simulink library "lib_SecCtrl_MASmsg"  (R2026a)
settings: Solver=VariableStepAuto
undefined symbols (not defined in the file): buses_lf, DiscIntNeverNeededParam, entity, iPs_lf, iQs_lf, last_send, m, Ps_lf, Qs_lf, set_DG_up, set_extra_satur, set_sending_cost, v_buses_mod
libraries: simulink x400, sl_discontinuities x10, eeGeneralControl x5
(part 7 of 12)

== system lib_SecCtrl_MASmsg/MAS messages/ID1/Simulink Function34 ==
  Input1 : Inport
  get_asked : TriggerPort  TriggerType=function-call  IsSimulinkFunction=on  FunctionName=get_asked  FunctionVisibility=scoped  VariantControl=(inherit)
  value : ArgOut  ArgumentName=value
  wires:
  Input1/1 -> value/1

== system lib_SecCtrl_MASmsg/MAS messages/ID1/Simulink Function35 ==
  Input : Inport
  get_extra_satur : TriggerPort  TriggerType=function-call  IsSimulinkFunction=on  FunctionName=get_extra_satur  FunctionVisibility=scoped  VariantControl=(inherit)
  y : ArgOut  ArgumentName=y
  wires:
  Input/1 -> y/1

== system lib_SecCtrl_MASmsg/MAS messages/ID1/Simulink Function36 ==
  Input1 : Inport
  get_Opt : TriggerPort  TriggerType=function-call  IsSimulinkFunction=on  FunctionName=get_Opt  FunctionVisibility=scoped  VariantControl=(inherit)
  value : ArgOut  ArgumentName=value
  wires:
  Input1/1 -> value/1

== system lib_SecCtrl_MASmsg/MAS messages/ID1/Simulink Function37 ==
  set_sending_cost : TriggerPort  TriggerType=function-call  IsSimulinkFunction=on  FunctionName=set_sending_cost  FunctionVisibility=scoped  VariantControl=(inherit)
  u : ArgIn  DisableCoverage=on  ArgumentName=u
  Output : Outport
  wires:
  u/1 -> Output/1

== system lib_SecCtrl_MASmsg/MAS messages/ID1/Simulink Function38 ==
  set_extra_satur : TriggerPort  TriggerType=function-call  IsSimulinkFunction=on  FunctionName=set_extra_satur  FunctionVisibility=scoped  VariantControl=(inherit)
  u : ArgIn  DisableCoverage=on  ArgumentName=u
  Output : Outport
  wires:
  u/1 -> Output/1

== system lib_SecCtrl_MASmsg/MAS messages/ID1/Simulink Function4 ==
  Input2 : Inport
  last_send : TriggerPort  TriggerType=function-call  IsSimulinkFunction=on  FunctionName=last_send  FunctionVisibility=scoped  VariantControl=(inherit)
  u : ArgIn  DisableCoverage=on  ArgumentName=v
  u1 : ArgIn  DisableCoverage=on  Port=2  ArgumentName=omega
  Output : Outport
  Output1 : Outport  Port=2
  time : Outport  Port=3
  wires:
  u/1 -> Output/1  "v"
  u1/1 -> Output1/1  "omega"
  Input2/1 -> time/1  "time"

== system lib_SecCtrl_MASmsg/MAS messages/ID1/Simulink Function5 ==
  send_to : TriggerPort  TriggerType=function-call  IsSimulinkFunction=on  FunctionName=send_to  FunctionVisibility=scoped  VariantControl=(inherit)
  u : ArgIn  DisableCoverage=on  ArgumentName=u
  Output : Outport
  wires:
  u/1 -> Output/1

== system lib_SecCtrl_MASmsg/MAS messages/ID1/Simulink Function6 ==
  Input1 : Inport
  Dest : TriggerPort  TriggerType=function-call  IsSimulinkFunction=on  FunctionName=Dest  FunctionVisibility=scoped  VariantControl=(inherit)
  Dest~ : ArgOut  DisableCoverage=on  ArgumentName=Dest
  wires:
  Input1/1 -> Dest~/1  "Dest"

== system lib_SecCtrl_MASmsg/MAS messages/ID1/Simulink Function7 ==
  set_following : TriggerPort  TriggerType=function-call  IsSimulinkFunction=on  FunctionName=set_following  FunctionVisibility=scoped  VariantControl=(inherit)
  u : ArgIn  DisableCoverage=on  ArgumentName=u
  Output : Outport
  wires:
  u/1 -> Output/1

== system lib_SecCtrl_MASmsg/MAS messages/ID1/Simulink Function8 ==
  type : TriggerPort  TriggerType=function-call  IsSimulinkFunction=on  FunctionName=type  FunctionVisibility=scoped  VariantControl=(inherit)
  Compare To Constant : simulink/Logic and Bit Operations/Compare To Constant  relop=~=  const=0  OutDataTypeStr=boolean  ZeroCross=off
  Send : Send  OutputPortMessageModes=m  ShowEnablePort=on
      settings: InputPortMap=e0,u1
  u : ArgIn  DisableCoverage=on  ArgumentName=u
  type_out : Outport
  trigger : Outport  Port=2
  wires:
  u/1 -> Compare To Constant/1, type_out/1
  Compare To Constant/1 -> Send/1, Send/2
  Send/1 -> trigger/1

== system lib_SecCtrl_MASmsg/MAS messages/ID1/Simulink Function9 ==
  Input1 : Inport
  get_leader : TriggerPort  TriggerType=function-call  IsSimulinkFunction=on  FunctionName=get_leader  FunctionVisibility=scoped  VariantControl=(inherit)
  value : ArgOut  ArgumentName=value
  wires:
  Input1/1 -> value/1

== system lib_SecCtrl_MASmsg/MAS messages/ID1/Subsystem ==
  In1 : Inport
  In3 : Inport  Port=2
  In4 : Inport  Port=3
  AND11 : Logic  IconShape=distinctive  AllPortsSameDT=off  OutDataTypeStr=boolean
  AND9 : Logic  IconShape=distinctive  AllPortsSameDT=off  OutDataTypeStr=boolean
  Compare To Zero : simulink/Logic and Bit Operations/Compare To Zero  relop=>  OutDataTypeStr=boolean
  Compare To Zero1 : simulink/Logic and Bit Operations/Compare To Zero  relop=<  OutDataTypeStr=boolean
  NOT : Logic  Operator=NOT  IconShape=distinctive  AllPortsSameDT=off  OutDataTypeStr=boolean
  OR4 : Logic  Operator=OR  IconShape=distinctive  AllPortsSameDT=off  OutDataTypeStr=boolean
  Relational Operator2 : RelationalOperator  Operator=<  OutDataTypeStr=boolean  RndMeth=Simplest  InputSameDT=off
  Relational Operator3 : RelationalOperator  Operator=>  OutDataTypeStr=boolean  RndMeth=Simplest  InputSameDT=off
  Out1 : Outport
  inf_satur : Outport  Port=2
  wires:
  NOT/1 -> Out1/1
  Compare To Zero/1 -> AND9/2
  Compare To Zero1/1 -> AND11/2
  In3/1 -> Relational Operator3/2, Relational Operator2/2
  Relational Operator3/1 -> AND11/1
  AND11/1 -> OR4/2, inf_satur/1
  In4/1 -> Relational Operator3/1, Relational Operator2/1
  AND9/1 -> OR4/1
  Relational Operator2/1 -> AND9/1
  OR4/1 -> NOT/1
  In1/1 -> Compare To Zero1/1, Compare To Zero/1

== system lib_SecCtrl_MASmsg/MAS messages/ID1/Triggered Subsystem ==
  In1 : Inport
  Trigger : TriggerPort  VariantControl=(inherit)
  Out1 : Outport
  wires:
  In1/1 -> Out1/1

== system lib_SecCtrl_MASmsg/MAS messages/ID1/Triggered Subsystem1 ==
  In1 : Inport
  Trigger : TriggerPort  VariantControl=(inherit)
  Out1 : Outport
  wires:
  In1/1 -> Out1/1

== system lib_SecCtrl_MASmsg/MAS messages/ID1/Triggered Subsystem2 ==
  In1 : Inport
  Trigger : TriggerPort  VariantControl=(inherit)
  Out1 : Outport
  wires:
  In1/1 -> Out1/1

== system lib_SecCtrl_MASmsg/MAS messages/ID1/Triggered Subsystem3 ==
  Trigger : TriggerPort  VariantControl=(inherit)
  One : Constant  OutDataTypeStr=Inherit: Inherit via back propagation
  Send7 : Send  OutputPortMessageModes=m  ShowEnablePort=on
      settings: InputPortMap=e0,u1
  Out1 : Outport
  wires:
  One/1 -> Send7/1, Send7/2
  Send7/1 -> Out1/1

== system lib_SecCtrl_MASmsg/MAS messages/ID1/Triggered Subsystem4 ==
  In1 : Inport
  Trigger : TriggerPort  VariantControl=(inherit)
  Out1 : Outport
  wires:
  In1/1 -> Out1/1

== system lib_SecCtrl_MASmsg/MAS messages/ID1/Triggered Subsystem5 ==
  In1 : Inport
  Trigger : TriggerPort  TriggerType=falling  VariantControl=(inherit)
  Constant : Constant
  IC : InitialCondition  Value=0
  Out1 : Outport
  Output : Outport  Port=2
  wires:
  IC/1 -> Output/1
  Constant/1 -> IC/1
  In1/1 -> Out1/1

== system lib_SecCtrl_MASmsg/MAS messages/ID1/ramp ==
  connected : Inport
  time : Inport  Port=2
  Clock5 : Clock
      settings: DisableCoverage=on
  Gain : Gain  Gain=0.05
  Product : Product
  Sum6 : Sum  DisableCoverage=on  Inputs=|+-  InputSameDT=on  SaturateOnIntegerOverflow=on  OutDataTypeStr=Inherit: Same as first input
  Out1 : Outport
  wires:
  Clock5/1 -> Sum6/1
  time/1 -> Sum6/2
  Sum6/1 -> Product/2
  Gain/1 -> Out1/1
  Product/1 -> Gain/1
  connected/1 -> Product/1

== system lib_SecCtrl_MASmsg/MAS messages/ID1/time ==
  time : Inport
  Trigger : TriggerPort  VariantControl=(inherit)
  Out1 : Outport
  wires:
  time/1 -> Out1/1

== system lib_SecCtrl_MASmsg/MAS messages/ID2/Compare to last ==
  Output : Inport
  In4 : Inport  Port=2
  In1 : Inport  Port=3
  Output1 : Inport  Port=4
  time_last : Inport  Port=5
  com : Inport  Port=6
  AND : Logic  Inputs=3  IconShape=distinctive  AllPortsSameDT=off  OutDataTypeStr=boolean
  Abs : Abs  ZeroCross=off  SaturateOnIntegerOverflow=off
  Abs1 : Abs  ZeroCross=off  SaturateOnIntegerOverflow=off
  Clock1 : Clock
  Compare To Constant1 : simulink/Logic and Bit Operations/Compare To Constant  relop=>  const=1  OutDataTypeStr=boolean  ZeroCross=off
  Compare To Constant2 : simulink/Logic and Bit Operations/Compare To Constant  relop=>  const=1e-2  OutDataTypeStr=boolean  ZeroCross=off
  Gain : Gain  Gain=1e2
  Gain1 : Gain  Gain=1e2
  Send1 : Send  OutputPortMessageModes=m  ShowEnablePort=on
      settings: InputPortMap=e0,u1
  Sum : Sum  Inputs=|+-
  Sum1 : Sum  Inputs=|+-
  Sum2 : Sum  Inputs=|++
  Sum5 : Sum  Inputs=|+-
  Trigger : Outport
  wires:
  com/1 -> AND/3
  Gain1/1 -> Sum2/2
  Gain/1 -> Sum2/1
  Compare To Constant1/1 -> AND/1
  Sum2/1 -> Compare To Constant1/1
  Abs1/1 -> Gain1/1
  Compare To Constant2/1 -> AND/2
  Clock1/1 -> Sum1/1  "time"
  time_last/1 -> Sum1/2  "time_last"
  Sum1/1 -> Compare To Constant2/1
  AND/1 -> Send1/2, Send1/1
  In4/1 -> Sum5/2  "last_omega"
  Sum5/1 -> Abs1/1
  Abs/1 -> Gain/1
  Sum/1 -> Abs/1
  Send1/1 -> Trigger/1
  Output1/1 -> Sum5/1  "omega"
  In1/1 -> Sum/1  "v"
  Output/1 -> Sum/2  "last_v"

== system lib_SecCtrl_MASmsg/MAS messages/ID2/Send to neighbor ==
  note: 1) Add Subsystem or Model blocks as valid variant choices.
      | 2) You cannot connect blocks at this level. At simulation, connectivity is automatically
      | determined, based on the active variant and port name matching.
  Message : Inport
  five : Subsystem  VariantControl=five
  four : Subsystem  VariantControl=four
  one : Subsystem  VariantControl=one
  three : Subsystem  VariantControl=three
  two : Subsystem  VariantControl=two

== system lib_SecCtrl_MASmsg/MAS messages/ID2/Send to neighbor1 ==
  note: 1) Add Subsystem or Model blocks as valid variant choices.
      | 2) You cannot connect blocks at this level. At simulation, connectivity is automatically
      | determined, based on the active variant and port name matching.
  Message : Inport
  five : Subsystem  VariantControl=five
  four : Subsystem  VariantControl=four
  one : Subsystem  VariantControl=one
  three : Subsystem  VariantControl=three
  two : Subsystem  VariantControl=two

== system lib_SecCtrl_MASmsg/MAS messages/ID2/Send to neighbor2 ==
  note: 1) Add Subsystem or Model blocks as valid variant choices.
      | 2) You cannot connect blocks at this level. At simulation, connectivity is automatically
      | determined, based on the active variant and port name matching.
  Message : Inport
  five : Subsystem  VariantControl=five
  four : Subsystem  VariantControl=four
  one : Subsystem  VariantControl=one
  three : Subsystem  VariantControl=three
  two : Subsystem  VariantControl=two

== system lib_SecCtrl_MASmsg/MAS messages/ID2/Simulink Function ==
  Input : Inport
  get_cost : TriggerPort  TriggerType=function-call  IsSimulinkFunction=on  FunctionName=get_cost  FunctionVisibility=scoped  VariantControl=(inherit)
  y : ArgOut  DisableCoverage=on  ArgumentName=y
  wires:
  Input/1 -> y/1

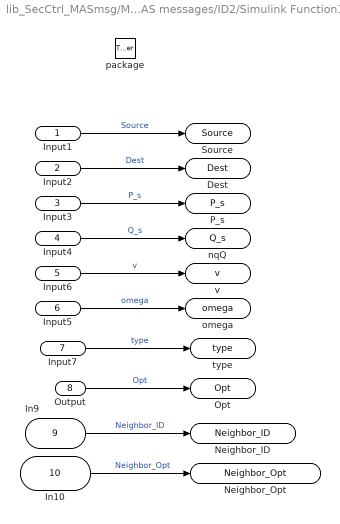
== system lib_SecCtrl_MASmsg/MAS messages/ID2/Simulink Function1 ==
  Input1 : Inport
  Input2 : Inport  Port=2
  Input3 : Inport  Port=3
  Input4 : Inport  Port=4
  Input6 : Inport  Port=5
  Input5 : Inport  Port=6
  Input7 : Inport  Port=7
  Output : Inport  Port=8
  In9 : Inport  Port=9
  In10 : Inport  Port=10
  package : TriggerPort  TriggerType=function-call  IsSimulinkFunction=on  FunctionName=package  FunctionVisibility=scoped  VariantControl=(inherit)
  Source : ArgOut  DisableCoverage=on  ArgumentName=Source
  Dest : ArgOut  DisableCoverage=on  Port=2  ArgumentName=Dest
  P_s : ArgOut  DisableCoverage=on  Port=3  ArgumentName=P_s
  nqQ : ArgOut  DisableCoverage=on  Port=4  ArgumentName=Q_s
  v : ArgOut  DisableCoverage=on  Port=5  ArgumentName=v
  omega : ArgOut  DisableCoverage=on  Port=6  ArgumentName=omega
  type : ArgOut  DisableCoverage=on  Port=7  ArgumentName=type
  Opt : ArgOut  Port=8  ArgumentName=Opt
  Neighbor_ID : ArgOut  Port=9  ArgumentName=Neighbor_ID
  Neighbor_Opt : ArgOut  Port=10  ArgumentName=Neighbor_Opt
  wires:
  In9/1 -> Neighbor_ID/1  "Neighbor_ID"
  In10/1 -> Neighbor_Opt/1  "Neighbor_Opt"
  Output/1 -> Opt/1  "Opt"
  Input7/1 -> type/1  "type"
  Input5/1 -> omega/1  "omega"
  Input6/1 -> v/1  "v"
  Input4/1 -> nqQ/1  "Q_s"
  Input3/1 -> P_s/1  "P_s"
  Input2/1 -> Dest/1  "Dest"
  Input1/1 -> Source/1  "Source"

== system lib_SecCtrl_MASmsg/MAS messages/ID2/Simulink Function10 ==
  set_leader : TriggerPort  TriggerType=function-call  IsSimulinkFunction=on  FunctionName=set_leader  FunctionVisibility=scoped  VariantControl=(inherit)
  u : ArgIn  DisableCoverage=on  ArgumentName=u
  Output : Outport
  wires:
  u/1 -> Output/1

== system lib_SecCtrl_MASmsg/MAS messages/ID2/Simulink Function11 ==
  Input1 : Inport
  get_sending : TriggerPort  TriggerType=function-call  IsSimulinkFunction=on  FunctionName=get_sending  FunctionVisibility=scoped  VariantControl=(inherit)
  value : ArgOut  ArgumentName=value
  wires:
  Input1/1 -> value/1

== system lib_SecCtrl_MASmsg/MAS messages/ID2/Simulink Function12 ==
  set_sending : TriggerPort  TriggerType=function-call  IsSimulinkFunction=on  FunctionName=set_sending  FunctionVisibility=scoped  VariantControl=(inherit)
  u : ArgIn  DisableCoverage=on  ArgumentName=u
  Output : Outport
  wires:
  u/1 -> Output/1

== system lib_SecCtrl_MASmsg/MAS messages/ID2/Simulink Function13 ==
  Input1 : Inport
  get_type : TriggerPort  TriggerType=function-call  IsSimulinkFunction=on  FunctionName=get_type  FunctionVisibility=scoped  VariantControl=(inherit)
  value : ArgOut  ArgumentName=type
  wires:
  Input1/1 -> value/1  "type"

== system lib_SecCtrl_MASmsg/MAS messages/ID2/Simulink Function14 ==
  set_cost_info : TriggerPort  TriggerType=function-call  IsSimulinkFunction=on  FunctionName=set_cost_info  FunctionVisibility=scoped  VariantControl=(inherit)
  cost : ArgIn  ArgumentName=cost
  Output : Outport
  wires:
  cost/1 -> Output/1

== system lib_SecCtrl_MASmsg/MAS messages/ID2/Simulink Function15 ==
  set_DG_up : TriggerPort  TriggerType=function-call  IsSimulinkFunction=on  FunctionName=set_DG_up  FunctionVisibility=scoped  VariantControl=(inherit)
  u : ArgIn  DisableCoverage=on  ArgumentName=u
  Output : Outport
  wires:
  u/1 -> Output/1

== system lib_SecCtrl_MASmsg/MAS messages/ID2/Simulink Function16 ==
  Input1 : Inport
  get_DG_up : TriggerPort  TriggerType=function-call  IsSimulinkFunction=on  FunctionName=get_DG_up  FunctionVisibility=scoped  VariantControl=(inherit)
  value : ArgOut  OutDataTypeStr=boolean  ArgumentName=value
  wires:
  Input1/1 -> value/1

== system lib_SecCtrl_MASmsg/MAS messages/ID2/Simulink Function17 ==
  set_neigh_ID : TriggerPort  TriggerType=function-call  IsSimulinkFunction=on  FunctionName=set_neigh_ID  FunctionVisibility=scoped  VariantControl=(inherit)
  u : ArgIn  DisableCoverage=on  ArgumentName=u
  Output : Outport
  wires:
  u/1 -> Output/1

== system lib_SecCtrl_MASmsg/MAS messages/ID2/Simulink Function18 ==
  Input1 : Inport
  get_neigh_ID : TriggerPort  TriggerType=function-call  IsSimulinkFunction=on  FunctionName=get_neigh_ID  FunctionVisibility=scoped  VariantControl=(inherit)
  value : ArgOut  ArgumentName=value
  wires:
  Input1/1 -> value/1

== system lib_SecCtrl_MASmsg/MAS messages/ID2/Simulink Function19 ==
  set_neigh_Opt : TriggerPort  TriggerType=function-call  IsSimulinkFunction=on  FunctionName=set_neigh_Opt  FunctionVisibility=scoped  VariantControl=(inherit)
  u : ArgIn  DisableCoverage=on  ArgumentName=u
  Output : Outport
  wires:
  u/1 -> Output/1

== system lib_SecCtrl_MASmsg/MAS messages/ID2/Simulink Function2 ==
  unpackage : TriggerPort  TriggerType=function-call  IsSimulinkFunction=on  FunctionName=unpackage  FunctionVisibility=scoped  VariantControl=(inherit)
  IC1 : InitialCondition
  IC2 : InitialCondition
  IC3 : InitialCondition  Value=v_buses_mod(buses_lf(IDnumber))
  IC4 : InitialCondition
  mpP~ : ArgIn  ArgumentName=P_s
  nqQ~ : ArgIn  Port=2  ArgumentName=Q_s
  v : ArgIn  Port=3  ArgumentName=v
  omega : ArgIn  Port=4  ArgumentName=omega
  Output2 : Outport
  Output3 : Outport  Port=2
  Output4 : Outport  Port=3
  Output5 : Outport  Port=4
  wires:
  omega/1 -> IC4/1  "omega"
  v/1 -> IC3/1  "v"
  nqQ~/1 -> IC2/1  "Q_s"
  mpP~/1 -> IC1/1  "P_s"
  IC1/1 -> Output2/1
  IC2/1 -> Output3/1
  IC4/1 -> Output5/1
  IC3/1 -> Output4/1

== system lib_SecCtrl_MASmsg/MAS messages/ID2/Simulink Function20 ==
  Input1 : Inport
  get_neigh_Opt : TriggerPort  TriggerType=function-call  IsSimulinkFunction=on  FunctionName=get_neigh_Opt  FunctionVisibility=scoped  VariantControl=(inherit)
  value : ArgOut  ArgumentName=value
  wires:
  Input1/1 -> value/1

== system lib_SecCtrl_MASmsg/MAS messages/ID2/Simulink Function21 ==
  set_sum_neigh_left : TriggerPort  TriggerType=function-call  IsSimulinkFunction=on  FunctionName=set_sum_neigh_left  FunctionVisibility=scoped  VariantControl=(inherit)
  u : ArgIn  DisableCoverage=on  ArgumentName=u
  Output : Outport
  wires:
  u/1 -> Output/1

== system lib_SecCtrl_MASmsg/MAS messages/ID2/Simulink Function22 ==
  set_Opt : TriggerPort  TriggerType=function-call  IsSimulinkFunction=on  FunctionName=set_Opt  FunctionVisibility=scoped  VariantControl=(inherit)
  u : ArgIn  DisableCoverage=on  ArgumentName=u
  Output : Outport
  wires:
  u/1 -> Output/1

== system lib_SecCtrl_MASmsg/MAS messages/ID2/Simulink Function23 ==
  Input1 : Inport
  get_sum_neigh_left : TriggerPort  TriggerType=function-call  IsSimulinkFunction=on  FunctionName=get_sum_neigh_left  FunctionVisibility=scoped  VariantControl=(inherit)
  value : ArgOut  ArgumentName=value
  wires:
  Input1/1 -> value/1  "sum_neigh_left"

== system lib_SecCtrl_MASmsg/MAS messages/ID2/Simulink Function24 ==
  set_decision_turn : TriggerPort  TriggerType=function-call  IsSimulinkFunction=on  FunctionName=set_decision_turn  FunctionVisibility=scoped  VariantControl=(inherit)
  u : ArgIn  DisableCoverage=on  ArgumentName=u
  Output : Outport
  wires:
  u/1 -> Output/1

== system lib_SecCtrl_MASmsg/MAS messages/ID2/Simulink Function25 ==
  Input1 : Inport
  get_ID : TriggerPort  TriggerType=function-call  IsSimulinkFunction=on  FunctionName=get_ID  FunctionVisibility=scoped  VariantControl=(inherit)
  value : ArgOut  ArgumentName=value
  wires:
  Input1/1 -> value/1

== system lib_SecCtrl_MASmsg/MAS messages/ID2/Simulink Function26 ==
  set_Neighbor_ID : TriggerPort  TriggerType=function-call  IsSimulinkFunction=on  FunctionName=set_Neighbor_ID  FunctionVisibility=scoped  VariantControl=(inherit)
  u : ArgIn  DisableCoverage=on  ArgumentName=u
  Output : Outport
  wires:
  u/1 -> Output/1

== system lib_SecCtrl_MASmsg/MAS messages/ID2/Simulink Function27 ==
  set_original_Opt : TriggerPort  TriggerType=function-call  IsSimulinkFunction=on  FunctionName=set_original_Opt  FunctionVisibility=scoped  VariantControl=(inherit)
  u : ArgIn  DisableCoverage=on  ArgumentName=u
  Output : Outport
  wires:
  u/1 -> Output/1

== system lib_SecCtrl_MASmsg/MAS messages/ID2/Simulink Function28 ==
  set_Neighbor_Opt : TriggerPort  TriggerType=function-call  IsSimulinkFunction=on  FunctionName=set_Neighbor_Opt  FunctionVisibility=scoped  VariantControl=(inherit)
  u : ArgIn  DisableCoverage=on  ArgumentName=u
  Output : Outport
  wires:
  u/1 -> Output/1

== system lib_SecCtrl_MASmsg/MAS messages/ID2/Simulink Function29 ==
  Input1 : Inport
  get_original_Opt : TriggerPort  TriggerType=function-call  IsSimulinkFunction=on  FunctionName=get_original_Opt  FunctionVisibility=scoped  VariantControl=(inherit)
  value : ArgOut  ArgumentName=value
  wires:
  Input1/1 -> value/1

== system lib_SecCtrl_MASmsg/MAS messages/ID2/Simulink Function3 ==
  Input1 : Inport
  get_following : TriggerPort  TriggerType=function-call  IsSimulinkFunction=on  FunctionName=get_following  FunctionVisibility=scoped  VariantControl=(inherit)
  value : ArgOut  ArgumentName=value
  wires:
  Input1/1 -> value/1

== system lib_SecCtrl_MASmsg/MAS messages/ID2/Simulink Function30 ==
  set_original_ID : TriggerPort  TriggerType=function-call  IsSimulinkFunction=on  FunctionName=set_original_ID  FunctionVisibility=scoped  VariantControl=(inherit)
  u : ArgIn  DisableCoverage=on  ArgumentName=u
  Output : Outport
  wires:
  u/1 -> Output/1

== system lib_SecCtrl_MASmsg/MAS messages/ID2/Simulink Function31 ==
  Input1 : Inport
  get_original_ID : TriggerPort  TriggerType=function-call  IsSimulinkFunction=on  FunctionName=get_original_ID  FunctionVisibility=scoped  VariantControl=(inherit)
  value : ArgOut  ArgumentName=value
  wires:
  Input1/1 -> value/1

== system lib_SecCtrl_MASmsg/MAS messages/ID2/Simulink Function32 ==
  set_asked : TriggerPort  TriggerType=function-call  IsSimulinkFunction=on  FunctionName=set_asked  FunctionVisibility=scoped  VariantControl=(inherit)
  u : ArgIn  DisableCoverage=on  ArgumentName=u
  Output : Outport
  wires:
  u/1 -> Output/1

== system lib_SecCtrl_MASmsg/MAS messages/ID2/Simulink Function33 ==
  Input : Inport
  get_cost_P : TriggerPort  TriggerType=function-call  IsSimulinkFunction=on  FunctionName=get_cost_P  FunctionVisibility=scoped  VariantControl=(inherit)
  y : ArgOut  DisableCoverage=on  ArgumentName=y
  wires:
  Input/1 -> y/1

== system lib_SecCtrl_MASmsg/MAS messages/ID2/Simulink Function34 ==
  Input1 : Inport
  get_asked : TriggerPort  TriggerType=function-call  IsSimulinkFunction=on  FunctionName=get_asked  FunctionVisibility=scoped  VariantControl=(inherit)
  value : ArgOut  ArgumentName=value
  wires:
  Input1/1 -> value/1

== system lib_SecCtrl_MASmsg/MAS messages/ID2/Simulink Function35 ==
  Input : Inport
  get_extra_satur : TriggerPort  TriggerType=function-call  IsSimulinkFunction=on  FunctionName=get_extra_satur  FunctionVisibility=scoped  VariantControl=(inherit)
  y : ArgOut  ArgumentName=y
  wires:
  Input/1 -> y/1

== system lib_SecCtrl_MASmsg/MAS messages/ID2/Simulink Function36 ==
  Input1 : Inport
  get_Opt : TriggerPort  TriggerType=function-call  IsSimulinkFunction=on  FunctionName=get_Opt  FunctionVisibility=scoped  VariantControl=(inherit)
  value : ArgOut  ArgumentName=value
  wires:
  Input1/1 -> value/1

== system lib_SecCtrl_MASmsg/MAS messages/ID2/Simulink Function37 ==
  set_sending_cost : TriggerPort  TriggerType=function-call  IsSimulinkFunction=on  FunctionName=set_sending_cost  FunctionVisibility=scoped  VariantControl=(inherit)
  u : ArgIn  DisableCoverage=on  ArgumentName=u
  Output : Outport
  wires:
  u/1 -> Output/1

== system lib_SecCtrl_MASmsg/MAS messages/ID2/Simulink Function38 ==
  set_extra_satur : TriggerPort  TriggerType=function-call  IsSimulinkFunction=on  FunctionName=set_extra_satur  FunctionVisibility=scoped  VariantControl=(inherit)
  u : ArgIn  DisableCoverage=on  ArgumentName=u
  Output : Outport
  wires:
  u/1 -> Output/1

== system lib_SecCtrl_MASmsg/MAS messages/ID2/Simulink Function4 ==
  Input2 : Inport
  last_send : TriggerPort  TriggerType=function-call  IsSimulinkFunction=on  FunctionName=last_send  FunctionVisibility=scoped  VariantControl=(inherit)
  u : ArgIn  DisableCoverage=on  ArgumentName=v
  u1 : ArgIn  DisableCoverage=on  Port=2  ArgumentName=omega
  Output : Outport
  Output1 : Outport  Port=2
  time : Outport  Port=3
  wires:
  Input2/1 -> time/1  "time"
  u1/1 -> Output1/1  "omega"
  u/1 -> Output/1  "v"

== system lib_SecCtrl_MASmsg/MAS messages/ID2/Simulink Function5 ==
  send_to : TriggerPort  TriggerType=function-call  IsSimulinkFunction=on  FunctionName=send_to  FunctionVisibility=scoped  VariantControl=(inherit)
  u : ArgIn  DisableCoverage=on  ArgumentName=u
  Output : Outport
  wires:
  u/1 -> Output/1

== system lib_SecCtrl_MASmsg/MAS messages/ID2/Simulink Function6 ==
  Input1 : Inport
  Dest : TriggerPort  TriggerType=function-call  IsSimulinkFunction=on  FunctionName=Dest  FunctionVisibility=scoped  VariantControl=(inherit)
  Dest~ : ArgOut  DisableCoverage=on  ArgumentName=Dest
  wires:
  Input1/1 -> Dest~/1  "Dest"

== system lib_SecCtrl_MASmsg/MAS messages/ID2/Simulink Function7 ==
  set_following : TriggerPort  TriggerType=function-call  IsSimulinkFunction=on  FunctionName=set_following  FunctionVisibility=scoped  VariantControl=(inherit)
  u : ArgIn  DisableCoverage=on  ArgumentName=u
  Output : Outport
  wires:
  u/1 -> Output/1

== system lib_SecCtrl_MASmsg/MAS messages/ID2/Simulink Function8 ==
  type : TriggerPort  TriggerType=function-call  IsSimulinkFunction=on  FunctionName=type  FunctionVisibility=scoped  VariantControl=(inherit)
  Compare To Constant : simulink/Logic and Bit Operations/Compare To Constant  relop=~=  const=0  OutDataTypeStr=boolean  ZeroCross=off
  Send : Send  OutputPortMessageModes=m  ShowEnablePort=on
      settings: InputPortMap=e0,u1
  u : ArgIn  DisableCoverage=on  ArgumentName=u
  type_out : Outport
  trigger : Outport  Port=2
  wires:
  Send/1 -> trigger/1
  Compare To Constant/1 -> Send/2, Send/1
  u/1 -> type_out/1, Compare To Constant/1

== system lib_SecCtrl_MASmsg/MAS messages/ID2/Simulink Function9 ==
  Input1 : Inport
  get_leader : TriggerPort  TriggerType=function-call  IsSimulinkFunction=on  FunctionName=get_leader  FunctionVisibility=scoped  VariantControl=(inherit)
  value : ArgOut  ArgumentName=value
  wires:
  Input1/1 -> value/1

== system lib_SecCtrl_MASmsg/MAS messages/ID2/Subsystem ==
  In1 : Inport
  In3 : Inport  Port=2
  In4 : Inport  Port=3
  AND11 : Logic  IconShape=distinctive  AllPortsSameDT=off  OutDataTypeStr=boolean
  AND9 : Logic  IconShape=distinctive  AllPortsSameDT=off  OutDataTypeStr=boolean
  Compare To Zero : simulink/Logic and Bit Operations/Compare To Zero  relop=>  OutDataTypeStr=boolean
  Compare To Zero1 : simulink/Logic and Bit Operations/Compare To Zero  relop=<  OutDataTypeStr=boolean
  NOT : Logic  Operator=NOT  IconShape=distinctive  AllPortsSameDT=off  OutDataTypeStr=boolean
  OR4 : Logic  Operator=OR  IconShape=distinctive  AllPortsSameDT=off  OutDataTypeStr=boolean
  Relational Operator2 : RelationalOperator  Operator=<  OutDataTypeStr=boolean  RndMeth=Simplest  InputSameDT=off
  Relational Operator3 : RelationalOperator  Operator=>  OutDataTypeStr=boolean  RndMeth=Simplest  InputSameDT=off
  Out1 : Outport
  inf_satur : Outport  Port=2
  wires:
  In1/1 -> Compare To Zero/1, Compare To Zero1/1
  OR4/1 -> NOT/1
  Relational Operator2/1 -> AND9/1
  AND9/1 -> OR4/1
  In4/1 -> Relational Operator2/1, Relational Operator3/1
  AND11/1 -> inf_satur/1, OR4/2
  Relational Operator3/1 -> AND11/1
  In3/1 -> Relational Operator2/2, Relational Operator3/2
  Compare To Zero1/1 -> AND11/2
  Compare To Zero/1 -> AND9/2
  NOT/1 -> Out1/1

== system lib_SecCtrl_MASmsg/MAS messages/ID2/Triggered Subsystem ==
  In1 : Inport
  Trigger : TriggerPort  VariantControl=(inherit)
  Out1 : Outport
  wires:
  In1/1 -> Out1/1

== system lib_SecCtrl_MASmsg/MAS messages/ID2/Triggered Subsystem1 ==
  In1 : Inport
  Trigger : TriggerPort  VariantControl=(inherit)
  Out1 : Outport
  wires:
  In1/1 -> Out1/1

== system lib_SecCtrl_MASmsg/MAS messages/ID2/Triggered Subsystem2 ==
  In1 : Inport
  Trigger : TriggerPort  VariantControl=(inherit)
  Out1 : Outport
  wires:
  In1/1 -> Out1/1

== system lib_SecCtrl_MASmsg/MAS messages/ID2/Triggered Subsystem3 ==
  Trigger : TriggerPort  VariantControl=(inherit)
  One : Constant  OutDataTypeStr=Inherit: Inherit via back propagation
  Send7 : Send  OutputPortMessageModes=m  ShowEnablePort=on
      settings: InputPortMap=e0,u1
  Out1 : Outport
  wires:
  Send7/1 -> Out1/1
  One/1 -> Send7/2, Send7/1

== system lib_SecCtrl_MASmsg/MAS messages/ID2/Triggered Subsystem4 ==
  In1 : Inport
  Trigger : TriggerPort  VariantControl=(inherit)
  Out1 : Outport
  wires:
  In1/1 -> Out1/1

== system lib_SecCtrl_MASmsg/MAS messages/ID2/Triggered Subsystem5 ==
  In1 : Inport
  Trigger : TriggerPort  TriggerType=falling  VariantControl=(inherit)
  Constant : Constant
  IC : InitialCondition  Value=0
  Out1 : Outport
  Output : Outport  Port=2
  wires:
  In1/1 -> Out1/1
  Constant/1 -> IC/1
  IC/1 -> Output/1

== system lib_SecCtrl_MASmsg/MAS messages/ID2/ramp ==
  connected : Inport
  time : Inport  Port=2
  Clock5 : Clock
      settings: DisableCoverage=on
  Gain : Gain  Gain=0.05
  Product : Product
  Sum6 : Sum  DisableCoverage=on  Inputs=|+-  InputSameDT=on  SaturateOnIntegerOverflow=on  OutDataTypeStr=Inherit: Same as first input
  Out1 : Outport
  wires:
  connected/1 -> Product/1
  Product/1 -> Gain/1
  Gain/1 -> Out1/1
  Sum6/1 -> Product/2
  time/1 -> Sum6/2
  Clock5/1 -> Sum6/1

== system lib_SecCtrl_MASmsg/MAS messages/ID2/time ==
  time : Inport
  Trigger : TriggerPort  VariantControl=(inherit)
  Out1 : Outport
  wires:
  time/1 -> Out1/1

== system lib_SecCtrl_MASmsg/MAS messages/ID3/Compare to last ==
  Output : Inport
  In4 : Inport  Port=2
  In1 : Inport  Port=3
  Output1 : Inport  Port=4
  time_last : Inport  Port=5
  com : Inport  Port=6
  AND : Logic  Inputs=3  IconShape=distinctive  AllPortsSameDT=off  OutDataTypeStr=boolean
  Abs : Abs  ZeroCross=off  SaturateOnIntegerOverflow=off
  Abs1 : Abs  ZeroCross=off  SaturateOnIntegerOverflow=off
  Clock1 : Clock
  Compare To Constant1 : simulink/Logic and Bit Operations/Compare To Constant  relop=>  const=1  OutDataTypeStr=boolean  ZeroCross=off
  Compare To Constant2 : simulink/Logic and Bit Operations/Compare To Constant  relop=>  const=1e-2  OutDataTypeStr=boolean  ZeroCross=off
  Gain : Gain  Gain=1e2
  Gain1 : Gain  Gain=1e2
  Send1 : Send  OutputPortMessageModes=m  ShowEnablePort=on
      settings: InputPortMap=e0,u1
  Sum : Sum  Inputs=|+-
  Sum1 : Sum  Inputs=|+-
  Sum2 : Sum  Inputs=|++
  Sum5 : Sum  Inputs=|+-
  Trigger : Outport
  wires:
  com/1 -> AND/3
  Gain1/1 -> Sum2/2
  Gain/1 -> Sum2/1
  Compare To Constant1/1 -> AND/1
  Sum2/1 -> Compare To Constant1/1
  Abs1/1 -> Gain1/1
  Compare To Constant2/1 -> AND/2
  Clock1/1 -> Sum1/1  "time"
  time_last/1 -> Sum1/2  "time_last"
  Sum1/1 -> Compare To Constant2/1
  AND/1 -> Send1/2, Send1/1
  In4/1 -> Sum5/2  "last_omega"
  Sum5/1 -> Abs1/1
  Abs/1 -> Gain/1
  Sum/1 -> Abs/1
  Send1/1 -> Trigger/1
  Output1/1 -> Sum5/1  "omega"
  In1/1 -> Sum/1  "v"
  Output/1 -> Sum/2  "last_v"

== system lib_SecCtrl_MASmsg/MAS messages/ID3/Send to neighbor ==
  note: 1) Add Subsystem or Model blocks as valid variant choices.
      | 2) You cannot connect blocks at this level. At simulation, connectivity is automatically
      | determined, based on the active variant and port name matching.
  Message : Inport
  five : Subsystem  VariantControl=five
  four : Subsystem  VariantControl=four
  one : Subsystem  VariantControl=one
  three : Subsystem  VariantControl=three
  two : Subsystem  VariantControl=two

== system lib_SecCtrl_MASmsg/MAS messages/ID3/Send to neighbor1 ==
  note: 1) Add Subsystem or Model blocks as valid variant choices.
      | 2) You cannot connect blocks at this level. At simulation, connectivity is automatically
      | determined, based on the active variant and port name matching.
  Message : Inport
  five : Subsystem  VariantControl=five
  four : Subsystem  VariantControl=four
  one : Subsystem  VariantControl=one
  three : Subsystem  VariantControl=three
  two : Subsystem  VariantControl=two

== system lib_SecCtrl_MASmsg/MAS messages/ID3/Send to neighbor2 ==
  note: 1) Add Subsystem or Model blocks as valid variant choices.
      | 2) You cannot connect blocks at this level. At simulation, connectivity is automatically
      | determined, based on the active variant and port name matching.
  Message : Inport
  five : Subsystem  VariantControl=five
  four : Subsystem  VariantControl=four
  one : Subsystem  VariantControl=one
  three : Subsystem  VariantControl=three
  two : Subsystem  VariantControl=two

== system lib_SecCtrl_MASmsg/MAS messages/ID3/Simulink Function ==
  Input : Inport
  get_cost : TriggerPort  TriggerType=function-call  IsSimulinkFunction=on  FunctionName=get_cost  FunctionVisibility=scoped  VariantControl=(inherit)
  y : ArgOut  DisableCoverage=on  ArgumentName=y
  wires:
  Input/1 -> y/1

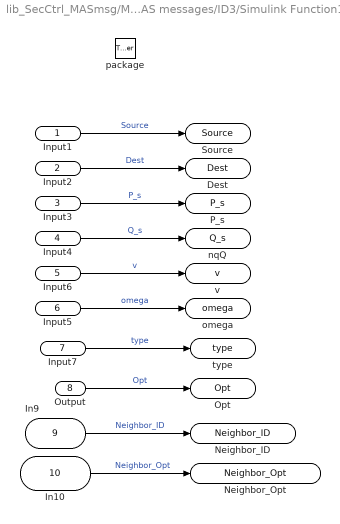
== system lib_SecCtrl_MASmsg/MAS messages/ID3/Simulink Function1 ==
  Input1 : Inport
  Input2 : Inport  Port=2
  Input3 : Inport  Port=3
  Input4 : Inport  Port=4
  Input6 : Inport  Port=5
  Input5 : Inport  Port=6
  Input7 : Inport  Port=7
  Output : Inport  Port=8
  In9 : Inport  Port=9
  In10 : Inport  Port=10
  package : TriggerPort  TriggerType=function-call  IsSimulinkFunction=on  FunctionName=package  FunctionVisibility=scoped  VariantControl=(inherit)
  Source : ArgOut  DisableCoverage=on  ArgumentName=Source
  Dest : ArgOut  DisableCoverage=on  Port=2  ArgumentName=Dest
  P_s : ArgOut  DisableCoverage=on  Port=3  ArgumentName=P_s
  nqQ : ArgOut  DisableCoverage=on  Port=4  ArgumentName=Q_s
  v : ArgOut  DisableCoverage=on  Port=5  ArgumentName=v
  omega : ArgOut  DisableCoverage=on  Port=6  ArgumentName=omega
  type : ArgOut  DisableCoverage=on  Port=7  ArgumentName=type
  Opt : ArgOut  Port=8  ArgumentName=Opt
  Neighbor_ID : ArgOut  Port=9  ArgumentName=Neighbor_ID
  Neighbor_Opt : ArgOut  Port=10  ArgumentName=Neighbor_Opt
  wires:
  In9/1 -> Neighbor_ID/1  "Neighbor_ID"
  In10/1 -> Neighbor_Opt/1  "Neighbor_Opt"
  Output/1 -> Opt/1  "Opt"
  Input7/1 -> type/1  "type"
  Input5/1 -> omega/1  "omega"
  Input6/1 -> v/1  "v"
  Input4/1 -> nqQ/1  "Q_s"
  Input3/1 -> P_s/1  "P_s"
  Input2/1 -> Dest/1  "Dest"
  Input1/1 -> Source/1  "Source"

== system lib_SecCtrl_MASmsg/MAS messages/ID3/Simulink Function10 ==
  set_leader : TriggerPort  TriggerType=function-call  IsSimulinkFunction=on  FunctionName=set_leader  FunctionVisibility=scoped  VariantControl=(inherit)
  u : ArgIn  DisableCoverage=on  ArgumentName=u
  Output : Outport
  wires:
  u/1 -> Output/1

== system lib_SecCtrl_MASmsg/MAS messages/ID3/Simulink Function11 ==
  Input1 : Inport
  get_sending : TriggerPort  TriggerType=function-call  IsSimulinkFunction=on  FunctionName=get_sending  FunctionVisibility=scoped  VariantControl=(inherit)
  value : ArgOut  ArgumentName=value
  wires:
  Input1/1 -> value/1

== system lib_SecCtrl_MASmsg/MAS messages/ID3/Simulink Function12 ==
  set_sending : TriggerPort  TriggerType=function-call  IsSimulinkFunction=on  FunctionName=set_sending  FunctionVisibility=scoped  VariantControl=(inherit)
  u : ArgIn  DisableCoverage=on  ArgumentName=u
  Output : Outport
  wires:
  u/1 -> Output/1

== system lib_SecCtrl_MASmsg/MAS messages/ID3/Simulink Function13 ==
  Input1 : Inport
  get_type : TriggerPort  TriggerType=function-call  IsSimulinkFunction=on  FunctionName=get_type  FunctionVisibility=scoped  VariantControl=(inherit)
  value : ArgOut  ArgumentName=type
  wires:
  Input1/1 -> value/1  "type"

== system lib_SecCtrl_MASmsg/MAS messages/ID3/Simulink Function14 ==
  set_cost_info : TriggerPort  TriggerType=function-call  IsSimulinkFunction=on  FunctionName=set_cost_info  FunctionVisibility=scoped  VariantControl=(inherit)
  cost : ArgIn  ArgumentName=cost
  Output : Outport
  wires:
  cost/1 -> Output/1

== system lib_SecCtrl_MASmsg/MAS messages/ID3/Simulink Function15 ==
  set_DG_up : TriggerPort  TriggerType=function-call  IsSimulinkFunction=on  FunctionName=set_DG_up  FunctionVisibility=scoped  VariantControl=(inherit)
  u : ArgIn  DisableCoverage=on  ArgumentName=u
  Output : Outport
  wires:
  u/1 -> Output/1

== system lib_SecCtrl_MASmsg/MAS messages/ID3/Simulink Function16 ==
  Input1 : Inport
  get_DG_up : TriggerPort  TriggerType=function-call  IsSimulinkFunction=on  FunctionName=get_DG_up  FunctionVisibility=scoped  VariantControl=(inherit)
  value : ArgOut  OutDataTypeStr=boolean  ArgumentName=value
  wires:
  Input1/1 -> value/1

== system lib_SecCtrl_MASmsg/MAS messages/ID3/Simulink Function17 ==
  set_neigh_ID : TriggerPort  TriggerType=function-call  IsSimulinkFunction=on  FunctionName=set_neigh_ID  FunctionVisibility=scoped  VariantControl=(inherit)
  u : ArgIn  DisableCoverage=on  ArgumentName=u
  Output : Outport
  wires:
  u/1 -> Output/1

== system lib_SecCtrl_MASmsg/MAS messages/ID3/Simulink Function18 ==
  Input1 : Inport
  get_neigh_ID : TriggerPort  TriggerType=function-call  IsSimulinkFunction=on  FunctionName=get_neigh_ID  FunctionVisibility=scoped  VariantControl=(inherit)
  value : ArgOut  ArgumentName=value
  wires:
  Input1/1 -> value/1

== system lib_SecCtrl_MASmsg/MAS messages/ID3/Simulink Function19 ==
  set_neigh_Opt : TriggerPort  TriggerType=function-call  IsSimulinkFunction=on  FunctionName=set_neigh_Opt  FunctionVisibility=scoped  VariantControl=(inherit)
  u : ArgIn  DisableCoverage=on  ArgumentName=u
  Output : Outport
  wires:
  u/1 -> Output/1

== system lib_SecCtrl_MASmsg/MAS messages/ID3/Simulink Function2 ==
  unpackage : TriggerPort  TriggerType=function-call  IsSimulinkFunction=on  FunctionName=unpackage  FunctionVisibility=scoped  VariantControl=(inherit)
  IC1 : InitialCondition
  IC2 : InitialCondition
  IC3 : InitialCondition  Value=v_buses_mod(buses_lf(IDnumber))
  IC4 : InitialCondition
  mpP~ : ArgIn  ArgumentName=P_s
  nqQ~ : ArgIn  Port=2  ArgumentName=Q_s
  v : ArgIn  Port=3  ArgumentName=v
  omega : ArgIn  Port=4  ArgumentName=omega
  Output2 : Outport
  Output3 : Outport  Port=2
  Output4 : Outport  Port=3
  Output5 : Outport  Port=4
  wires:
  omega/1 -> IC4/1  "omega"
  v/1 -> IC3/1  "v"
  nqQ~/1 -> IC2/1  "Q_s"
  mpP~/1 -> IC1/1  "P_s"
  IC1/1 -> Output2/1
  IC2/1 -> Output3/1
  IC4/1 -> Output5/1
  IC3/1 -> Output4/1

== system lib_SecCtrl_MASmsg/MAS messages/ID3/Simulink Function20 ==
  Input1 : Inport
  get_neigh_Opt : TriggerPort  TriggerType=function-call  IsSimulinkFunction=on  FunctionName=get_neigh_Opt  FunctionVisibility=scoped  VariantControl=(inherit)
  value : ArgOut  ArgumentName=value
  wires:
  Input1/1 -> value/1

== system lib_SecCtrl_MASmsg/MAS messages/ID3/Simulink Function21 ==
  set_sum_neigh_left : TriggerPort  TriggerType=function-call  IsSimulinkFunction=on  FunctionName=set_sum_neigh_left  FunctionVisibility=scoped  VariantControl=(inherit)
  u : ArgIn  DisableCoverage=on  ArgumentName=u
  Output : Outport
  wires:
  u/1 -> Output/1

== system lib_SecCtrl_MASmsg/MAS messages/ID3/Simulink Function22 ==
  set_Opt : TriggerPort  TriggerType=function-call  IsSimulinkFunction=on  FunctionName=set_Opt  FunctionVisibility=scoped  VariantControl=(inherit)
  u : ArgIn  DisableCoverage=on  ArgumentName=u
  Output : Outport
  wires:
  u/1 -> Output/1

== system lib_SecCtrl_MASmsg/MAS messages/ID3/Simulink Function23 ==
  Input1 : Inport
  get_sum_neigh_left : TriggerPort  TriggerType=function-call  IsSimulinkFunction=on  FunctionName=get_sum_neigh_left  FunctionVisibility=scoped  VariantControl=(inherit)
  value : ArgOut  ArgumentName=value
  wires:
  Input1/1 -> value/1  "sum_neigh_left"

== system lib_SecCtrl_MASmsg/MAS messages/ID3/Simulink Function24 ==
  set_decision_turn : TriggerPort  TriggerType=function-call  IsSimulinkFunction=on  FunctionName=set_decision_turn  FunctionVisibility=scoped  VariantControl=(inherit)
  u : ArgIn  DisableCoverage=on  ArgumentName=u
  Output : Outport
  wires:
  u/1 -> Output/1

== system lib_SecCtrl_MASmsg/MAS messages/ID3/Simulink Function25 ==
  Input1 : Inport
  get_ID : TriggerPort  TriggerType=function-call  IsSimulinkFunction=on  FunctionName=get_ID  FunctionVisibility=scoped  VariantControl=(inherit)
  value : ArgOut  ArgumentName=value
  wires:
  Input1/1 -> value/1

== system lib_SecCtrl_MASmsg/MAS messages/ID3/Simulink Function26 ==
  set_Neighbor_ID : TriggerPort  TriggerType=function-call  IsSimulinkFunction=on  FunctionName=set_Neighbor_ID  FunctionVisibility=scoped  VariantControl=(inherit)
  u : ArgIn  DisableCoverage=on  ArgumentName=u
  Output : Outport
  wires:
  u/1 -> Output/1

== system lib_SecCtrl_MASmsg/MAS messages/ID3/Simulink Function27 ==
  set_original_Opt : TriggerPort  TriggerType=function-call  IsSimulinkFunction=on  FunctionName=set_original_Opt  FunctionVisibility=scoped  VariantControl=(inherit)
  u : ArgIn  DisableCoverage=on  ArgumentName=u
  Output : Outport
  wires:
  u/1 -> Output/1

== system lib_SecCtrl_MASmsg/MAS messages/ID3/Simulink Function28 ==
  set_Neighbor_Opt : TriggerPort  TriggerType=function-call  IsSimulinkFunction=on  FunctionName=set_Neighbor_Opt  FunctionVisibility=scoped  VariantControl=(inherit)
  u : ArgIn  DisableCoverage=on  ArgumentName=u
  Output : Outport
  wires:
  u/1 -> Output/1

== system lib_SecCtrl_MASmsg/MAS messages/ID3/Simulink Function29 ==
  Input1 : Inport
  get_original_Opt : TriggerPort  TriggerType=function-call  IsSimulinkFunction=on  FunctionName=get_original_Opt  FunctionVisibility=scoped  VariantControl=(inherit)
  value : ArgOut  ArgumentName=value
  wires:
  Input1/1 -> value/1

== system lib_SecCtrl_MASmsg/MAS messages/ID3/Simulink Function3 ==
  Input1 : Inport
  get_following : TriggerPort  TriggerType=function-call  IsSimulinkFunction=on  FunctionName=get_following  FunctionVisibility=scoped  VariantControl=(inherit)
  value : ArgOut  ArgumentName=value
  wires:
  Input1/1 -> value/1

== system lib_SecCtrl_MASmsg/MAS messages/ID3/Simulink Function30 ==
  set_original_ID : TriggerPort  TriggerType=function-call  IsSimulinkFunction=on  FunctionName=set_original_ID  FunctionVisibility=scoped  VariantControl=(inherit)
  u : ArgIn  DisableCoverage=on  ArgumentName=u
  Output : Outport
  wires:
  u/1 -> Output/1

== system lib_SecCtrl_MASmsg/MAS messages/ID3/Simulink Function31 ==
  Input1 : Inport
  get_original_ID : TriggerPort  TriggerType=function-call  IsSimulinkFunction=on  FunctionName=get_original_ID  FunctionVisibility=scoped  VariantControl=(inherit)
  value : ArgOut  ArgumentName=value
  wires:
  Input1/1 -> value/1

== system lib_SecCtrl_MASmsg/MAS messages/ID3/Simulink Function32 ==
  set_asked : TriggerPort  TriggerType=function-call  IsSimulinkFunction=on  FunctionName=set_asked  FunctionVisibility=scoped  VariantControl=(inherit)
  u : ArgIn  DisableCoverage=on  ArgumentName=u
  Output : Outport
  wires:
  u/1 -> Output/1

== system lib_SecCtrl_MASmsg/MAS messages/ID3/Simulink Function33 ==
  Input : Inport
  get_cost_P : TriggerPort  TriggerType=function-call  IsSimulinkFunction=on  FunctionName=get_cost_P  FunctionVisibility=scoped  VariantControl=(inherit)
  y : ArgOut  DisableCoverage=on  ArgumentName=y
  wires:
  Input/1 -> y/1

== system lib_SecCtrl_MASmsg/MAS messages/ID3/Simulink Function34 ==
  Input1 : Inport
  get_asked : TriggerPort  TriggerType=function-call  IsSimulinkFunction=on  FunctionName=get_asked  FunctionVisibility=scoped  VariantControl=(inherit)
  value : ArgOut  ArgumentName=value
  wires:
  Input1/1 -> value/1

== system lib_SecCtrl_MASmsg/MAS messages/ID3/Simulink Function35 ==
  Input : Inport
  get_extra_satur : TriggerPort  TriggerType=function-call  IsSimulinkFunction=on  FunctionName=get_extra_satur  FunctionVisibility=scoped  VariantControl=(inherit)
  y : ArgOut  ArgumentName=y
  wires:
  Input/1 -> y/1

== system lib_SecCtrl_MASmsg/MAS messages/ID3/Simulink Function36 ==
  Input1 : Inport
  get_Opt : TriggerPort  TriggerType=function-call  IsSimulinkFunction=on  FunctionName=get_Opt  FunctionVisibility=scoped  VariantControl=(inherit)
  value : ArgOut  ArgumentName=value
  wires:
  Input1/1 -> value/1

== system lib_SecCtrl_MASmsg/MAS messages/ID3/Simulink Function37 ==
  set_sending_cost : TriggerPort  TriggerType=function-call  IsSimulinkFunction=on  FunctionName=set_sending_cost  FunctionVisibility=scoped  VariantControl=(inherit)
  u : ArgIn  DisableCoverage=on  ArgumentName=u
  Output : Outport
  wires:
  u/1 -> Output/1

== system lib_SecCtrl_MASmsg/MAS messages/ID3/Simulink Function38 ==
  set_extra_satur : TriggerPort  TriggerType=function-call  IsSimulinkFunction=on  FunctionName=set_extra_satur  FunctionVisibility=scoped  VariantControl=(inherit)
  u : ArgIn  DisableCoverage=on  ArgumentName=u
  Output : Outport
  wires:
  u/1 -> Output/1

== system lib_SecCtrl_MASmsg/MAS messages/ID3/Simulink Function4 ==
  Input2 : Inport
  last_send : TriggerPort  TriggerType=function-call  IsSimulinkFunction=on  FunctionName=last_send  FunctionVisibility=scoped  VariantControl=(inherit)
  u : ArgIn  DisableCoverage=on  ArgumentName=v
  u1 : ArgIn  DisableCoverage=on  Port=2  ArgumentName=omega
  Output : Outport
  Output1 : Outport  Port=2
  time : Outport  Port=3
  wires:
  Input2/1 -> time/1  "time"
  u1/1 -> Output1/1  "omega"
  u/1 -> Output/1  "v"

== system lib_SecCtrl_MASmsg/MAS messages/ID3/Simulink Function5 ==
  send_to : TriggerPort  TriggerType=function-call  IsSimulinkFunction=on  FunctionName=send_to  FunctionVisibility=scoped  VariantControl=(inherit)
  u : ArgIn  DisableCoverage=on  ArgumentName=u
  Output : Outport
  wires:
  u/1 -> Output/1

== system lib_SecCtrl_MASmsg/MAS messages/ID3/Simulink Function6 ==
  Input1 : Inport
  Dest : TriggerPort  TriggerType=function-call  IsSimulinkFunction=on  FunctionName=Dest  FunctionVisibility=scoped  VariantControl=(inherit)
  Dest~ : ArgOut  DisableCoverage=on  ArgumentName=Dest
  wires:
  Input1/1 -> Dest~/1  "Dest"

== system lib_SecCtrl_MASmsg/MAS messages/ID3/Simulink Function7 ==
  set_following : TriggerPort  TriggerType=function-call  IsSimulinkFunction=on  FunctionName=set_following  FunctionVisibility=scoped  VariantControl=(inherit)
  u : ArgIn  DisableCoverage=on  ArgumentName=u
  Output : Outport
  wires:
  u/1 -> Output/1

== system lib_SecCtrl_MASmsg/MAS messages/ID3/Simulink Function8 ==
  type : TriggerPort  TriggerType=function-call  IsSimulinkFunction=on  FunctionName=type  FunctionVisibility=scoped  VariantControl=(inherit)
  Compare To Constant : simulink/Logic and Bit Operations/Compare To Constant  relop=~=  const=0  OutDataTypeStr=boolean  ZeroCross=off
  Send : Send  OutputPortMessageModes=m  ShowEnablePort=on
      settings: InputPortMap=e0,u1
  u : ArgIn  DisableCoverage=on  ArgumentName=u
  type_out : Outport
  trigger : Outport  Port=2
  wires:
  Send/1 -> trigger/1
  Compare To Constant/1 -> Send/2, Send/1
  u/1 -> type_out/1, Compare To Constant/1

== system lib_SecCtrl_MASmsg/MAS messages/ID3/Simulink Function9 ==
  Input1 : Inport
  get_leader : TriggerPort  TriggerType=function-call  IsSimulinkFunction=on  FunctionName=get_leader  FunctionVisibility=scoped  VariantControl=(inherit)
  value : ArgOut  ArgumentName=value
  wires:
  Input1/1 -> value/1

== system lib_SecCtrl_MASmsg/MAS messages/ID3/Subsystem ==
  In1 : Inport
  In3 : Inport  Port=2
  In4 : Inport  Port=3
  AND11 : Logic  IconShape=distinctive  AllPortsSameDT=off  OutDataTypeStr=boolean
  AND9 : Logic  IconShape=distinctive  AllPortsSameDT=off  OutDataTypeStr=boolean
  Compare To Zero : simulink/Logic and Bit Operations/Compare To Zero  relop=>  OutDataTypeStr=boolean
  Compare To Zero1 : simulink/Logic and Bit Operations/Compare To Zero  relop=<  OutDataTypeStr=boolean
  NOT : Logic  Operator=NOT  IconShape=distinctive  AllPortsSameDT=off  OutDataTypeStr=boolean
  OR4 : Logic  Operator=OR  IconShape=distinctive  AllPortsSameDT=off  OutDataTypeStr=boolean
  Relational Operator2 : RelationalOperator  Operator=<  OutDataTypeStr=boolean  RndMeth=Simplest  InputSameDT=off
  Relational Operator3 : RelationalOperator  Operator=>  OutDataTypeStr=boolean  RndMeth=Simplest  InputSameDT=off
  Out1 : Outport
  inf_satur : Outport  Port=2
  wires:
  In1/1 -> Compare To Zero/1, Compare To Zero1/1
  OR4/1 -> NOT/1
  Relational Operator2/1 -> AND9/1
  AND9/1 -> OR4/1
  In4/1 -> Relational Operator2/1, Relational Operator3/1
  AND11/1 -> inf_satur/1, OR4/2
  Relational Operator3/1 -> AND11/1
  In3/1 -> Relational Operator2/2, Relational Operator3/2
  Compare To Zero1/1 -> AND11/2
  Compare To Zero/1 -> AND9/2
  NOT/1 -> Out1/1

== system lib_SecCtrl_MASmsg/MAS messages/ID3/Triggered Subsystem ==
  In1 : Inport
  Trigger : TriggerPort  VariantControl=(inherit)
  Out1 : Outport
  wires:
  In1/1 -> Out1/1

== system lib_SecCtrl_MASmsg/MAS messages/ID3/Triggered Subsystem1 ==
  In1 : Inport
  Trigger : TriggerPort  VariantControl=(inherit)
  Out1 : Outport
  wires:
  In1/1 -> Out1/1

== system lib_SecCtrl_MASmsg/MAS messages/ID3/Triggered Subsystem2 ==
  In1 : Inport
  Trigger : TriggerPort  VariantControl=(inherit)
  Out1 : Outport
  wires:
  In1/1 -> Out1/1

== system lib_SecCtrl_MASmsg/MAS messages/ID3/Triggered Subsystem3 ==
  Trigger : TriggerPort  VariantControl=(inherit)
  One : Constant  OutDataTypeStr=Inherit: Inherit via back propagation
  Send7 : Send  OutputPortMessageModes=m  ShowEnablePort=on
      settings: InputPortMap=e0,u1
  Out1 : Outport
  wires:
  Send7/1 -> Out1/1
  One/1 -> Send7/2, Send7/1

== system lib_SecCtrl_MASmsg/MAS messages/ID3/Triggered Subsystem4 ==
  In1 : Inport
  Trigger : TriggerPort  VariantControl=(inherit)
  Out1 : Outport
  wires:
  In1/1 -> Out1/1

== system lib_SecCtrl_MASmsg/MAS messages/ID3/Triggered Subsystem5 ==
  In1 : Inport
  Trigger : TriggerPort  TriggerType=falling  VariantControl=(inherit)
  Constant : Constant
  IC : InitialCondition  Value=0
  Out1 : Outport
  Output : Outport  Port=2
  wires:
  In1/1 -> Out1/1
  Constant/1 -> IC/1
  IC/1 -> Output/1

== system lib_SecCtrl_MASmsg/MAS messages/ID3/ramp ==
  connected : Inport
  time : Inport  Port=2
  Clock5 : Clock
      settings: DisableCoverage=on
  Gain : Gain  Gain=0.05
  Product : Product
  Sum6 : Sum  DisableCoverage=on  Inputs=|+-  InputSameDT=on  SaturateOnIntegerOverflow=on  OutDataTypeStr=Inherit: Same as first input
  Out1 : Outport
  wires:
  connected/1 -> Product/1
  Product/1 -> Gain/1
  Gain/1 -> Out1/1
  Sum6/1 -> Product/2
  time/1 -> Sum6/2
  Clock5/1 -> Sum6/1

== system lib_SecCtrl_MASmsg/MAS messages/ID3/time ==
  time : Inport
  Trigger : TriggerPort  VariantControl=(inherit)
  Out1 : Outport
  wires:
  time/1 -> Out1/1
